simulink model "simulation_2"  (R2026a)
settings: Solver=VariableStepAuto  StopTime=10000
undefined symbols (not defined in the file): battery_builder_rtmsupport, gcbh
libraries: fl_lib x3, nesl_utility x3, BatteryCurrentManagement x1, Batteries_lib x1, BatteryEstimators x1
settings Model: Creator=dom  LastModifiedBy=dom

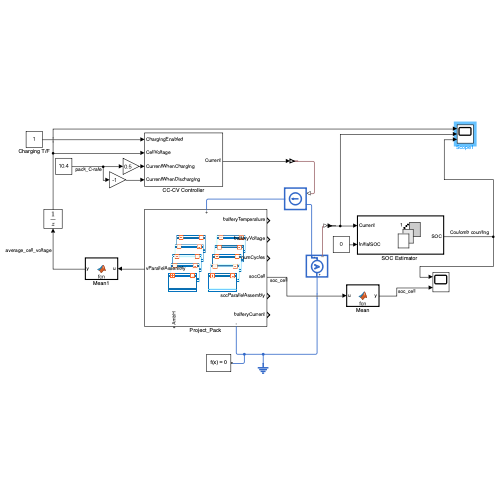
[thumbnail: Simulink's stored preview of the top-level diagram]
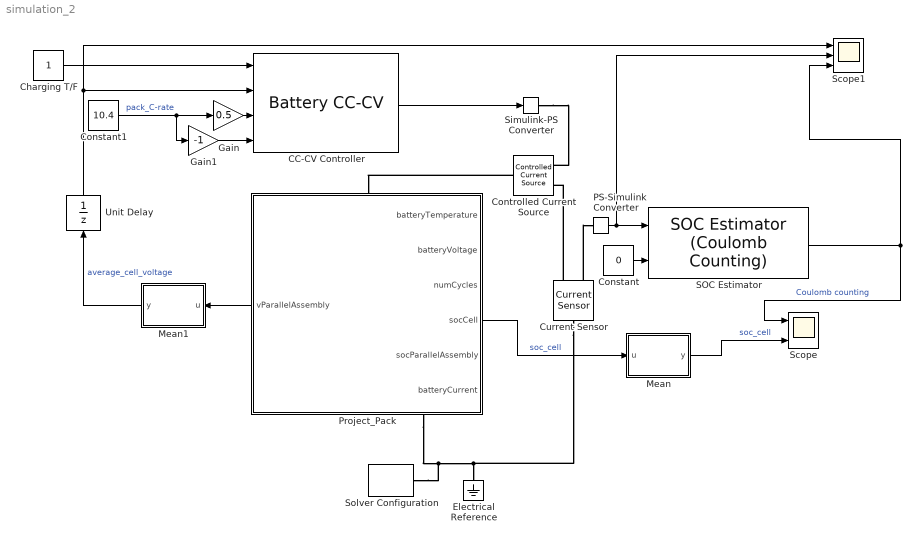
== system simulation_2 ==
  CC-CV Controller : BatteryCurrentManagement/Battery CC-CV  MinMaxFlag=off  MaxCellVoltage=4.2  Kp=100  Ki=10  Kaw=1  Kt=1  Ts=1
      settings: LibrarySourceBlock=batt_sl_lib/Current Management/Battery CC-CV
  Charging T/F : Constant
  Constant : Constant  Value=0
  Constant1 : Constant  Value=10.4
  Controlled Current Source : fl_lib/Electrical/Electrical Sources/Controlled Current Source
  Current Sensor : fl_lib/Electrical/Electrical Sensors/Current Sensor
  Electrical Reference : fl_lib/Electrical/Electrical Elements/Electrical Reference
  Gain : Gain  Gain=0.5
  Gain1 : Gain  Gain=-1
  Mean : MATLAB Function  TreatAsAtomicUnit=on
  Mean1 : MATLAB Function  TreatAsAtomicUnit=on
  PS-Simulink Converter : nesl_utility/PS-Simulink Converter  PhysicalDomain=network_engine_domain  SubClassName=ps_output  LeftPortType=input  RightPortType=output  PseudoPeriodic=off  Frequencies=[]  VectorFormat=inherit  Unit=inherit  AffineConversion=off
  Project_Pack : Subsystem  LoadFcn=battery_builder_rtmsupport('loadfcn',gcbh);
      settings: CopyFcn=battery_builder_rtmsupport('copyfcn',gcbh);  PreCopyFcn=battery_builder_rtmsupport('precopyfcn',gcbh);  PreDeleteFcn=battery_builder_rtmsupport('predeletefcn',gcbh);  PortSchema="{\"entries\":[{\"content\":{\"sides\":[{\"content\":{\"connectorIds\":[\"LConn1\"]},\"type\":\"ConnectorPlacement.EquallySpacedRectSide\",\"uuid\":\"76c6f046-db8e-4015-a922-00ba973faf16\"},{\"content\":{\"connectorIds\":[\"RConn1\",\"RConn2\"],\"side\":\"RIGHT\"},\"type\":\"ConnectorPlacement.EquallySpacedRectSide\",\"uuid\":\"59fdee5c-a6f4-4b44-aa6e-82d2d9418fce\"},{\"content\":{\"connectorIds\":[\"Out7\"],\"side\":\"TOP\"},\"type\":\"ConnectorPlacement.EquallySpacedRectSide\",\"uuid\":\"84b83595-cc1f-46da-a2b0-c16634a6daab\"},{\"content\":{\"connectorIds\":[\"Out1\",\"Out2\",\"Out3\",\"Out4\",\"Out5\",\"Out6\"],\"side\":\"BOTTOM\"},\"type\":\"ConnectorPlacement.EquallySpacedRectSide\",\"uuid\":\"4528fa0d-8164-4e66-baa6-2a345765de4f\"}]},\"type\":\"ConnectorPlacement.EquallySpacedConnector\",\"uuid\":\"e6fb231a-8daf-4bfc-bdc1-9175fa7a2dfd\"}],\"packageUris\":[\"http://schema.mathworks.com/mf0/Connector/R2020b\"],\"version\":\"1.0\"}"
      mask Display: image('$imagefile')
  "SOC Estimator " : BatteryEstimators/SOC Estimator (Coulomb Counting)  CurrentInputPartition=off  AH=10.4  Ts=1  DataType=Inherit: auto
      settings: LibrarySourceBlock=|
      | batt_sl_lib/Estimators/SOC Estimator
      | (Coulomb Counting)
  Scope : Scope  NumInputPorts=2
      settings: ActiveDisplayYMinimum=-0.12550450361997315  ActiveDisplayYMaximum=1.1295405325797585
  Scope1 : Scope  NumInputPorts=3
      settings: ActiveDisplayYMinimum=2.2867646550900531  ActiveDisplayYMaximum=4.4191181041895247
  Simulink-PS Converter : nesl_utility/Simulink-PS Converter  PhysicalDomain=network_engine_domain  SubClassName=ps_input  LeftPortType=input  RightPortType=output  PseudoPeriodic=off  Frequencies=[]  NoiseDistribution=none  NoiseParameters=[]  Unit=1  AffineConversion=off  FilteringAndDerivatives=provide  SimscapeFilterOrder=1  InputFilterTimeConstant=0.001  UdotUserProvided=0
  Solver Configuration : nesl_utility/Solver Configuration  PhysicalDomain=network_engine_domain  SubClassName=solver  LeftPortType=input  RightPortType=generic  Tones=[]  Harmonics=[]  SimulateNoise=off  Profile=off  UseLocalSampling=off  EnableSwitchedLinearOptims=on  FrequencyDomain=off  UseCCode=off  RelTol=0.001  AbsTol=0.001  MinStep=1e-09  ToWorkspace=off  RevertToSquareIcSolve=off  NumHomotopyIterations=100  PhasorMode=off  PhasorModeNumHarmonics=1  ConsistencySolver=NEWTON_XTOL_AFTER_FTOL  CanonicalOrdering=CANONICAL  OptimizeIntermediates=OPTIMIZED  IndexReductionMethod=DerivativeReplacement  DoDC=off  ResidualTolerance=1e-09  ConsistencyTolSource=GLOBAL  ConsistencyAbsTol=0.001  ConsistencyRelTol=0.001  ConsistencyTolFactor=0.001  UseLocalSolver=off  LocalSolverChoice=NE_BACKWARD_EULER_ADVANCER  ResolveIndetEquations=on  FunctionEvalNumThread=1  LocalSolverSampleTime=0.001  DoFixedCost=off  MaxNonlinIter=3  MaxModeIter=2  ComputeImpulses=off  ImpulseIterations=2  LinearAlgebra=auto  LinearAlgebraNumThread=0  EquationFormulation=NE_TIME_EF  DelaysMemoryBudget=1024  AutomaticFiltering=on  FilteringTimeConstant=0.001  PartitionStorageMethod=AS_NEEDED  PartitionMemoryBudget=1024  PartitionMethod=ROBUST  MultibodyUseLocalSolver=off  MultibodyLocalSolverChoice=ODE1  MultibodyLocalSolverSampleTime=0.001
  Unit Delay : UnitDelay  InitialCondition=2.5  SampleTime=-1
  wires:
  Project_Pack/4(socCell) -> Mean/1(u)  "soc_cell"
  Mean/1(y) -> Scope/2  "soc_cell"
  "SOC Estimator "/1 -> Scope/1, Scope1/3  "Coulomb counting"
  Constant/1 -> "SOC Estimator "/2
  PS-Simulink Converter/1 -> Scope1/2, "SOC Estimator "/1
  Gain/1 -> CC-CV Controller/3
  Project_Pack/7(vParallelAssembly) -> Mean1/1(u)
  Mean1/1(y) -> Unit Delay/1  "average_cell_voltage"
  Unit Delay/1 -> Scope1/1, CC-CV Controller/2
  Constant1/1 -> Gain/1, Gain1/1  "pack_C-rate"
  CC-CV Controller/1 -> Simulink-PS Converter/1
  Charging T/F/1 -> CC-CV Controller/1
  Gain1/1 -> CC-CV Controller/4
  connections:
  Project_Pack/RConn2 -- Current Sensor/LConn1 -- Electrical Reference/LConn1 -- Solver Configuration/RConn1
  Current Sensor/RConn1 -- PS-Simulink Converter/LConn1
  Simulink-PS Converter/RConn1 -- Controlled Current Source/RConn1
  Current Sensor/RConn2 -- Controlled Current Source/RConn2
  Controlled Current Source/LConn1 -- Project_Pack/LConn1

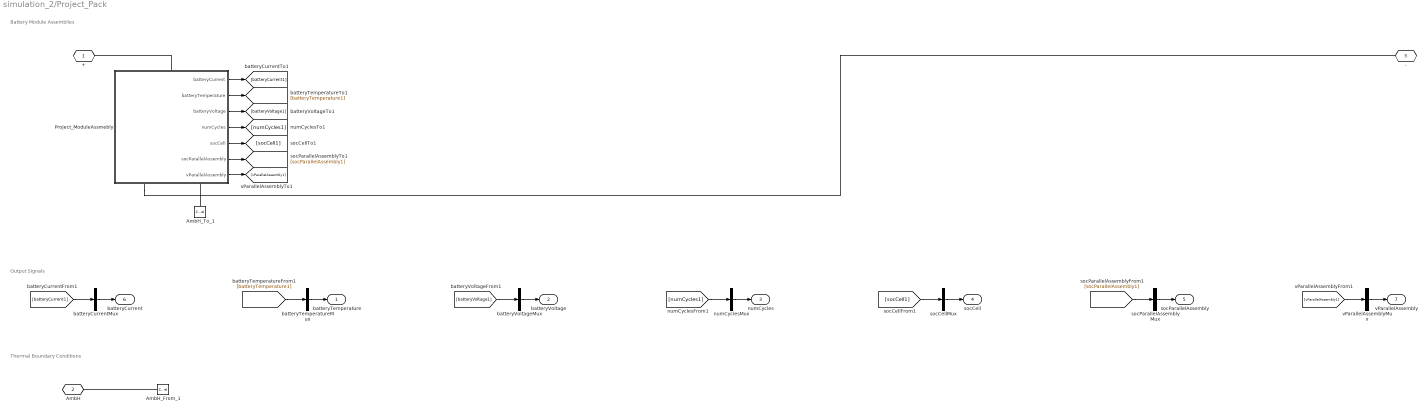
== system simulation_2/Project_Pack ==
  note: Thermal Boundary Conditions
  note: Output Signals
  note: Battery Module Assemblies
  AmbH_From_1 : ConnectionLabel  Label=ambH_1
  AmbH_To_1 : ConnectionLabel  Label=ambH_1
  Project_ModuleAssmebly : Subsystem  LoadFcn=battery_builder_rtmsupport('loadfcn',gcbh);
      settings: CopyFcn=battery_builder_rtmsupport('copyfcn',gcbh);  PreCopyFcn=battery_builder_rtmsupport('precopyfcn',gcbh);  PreDeleteFcn=battery_builder_rtmsupport('predeletefcn',gcbh);  PortSchema="{\"entries\":[{\"content\":{\"sides\":[{\"content\":{\"connectorIds\":[\"LConn1\"]},\"type\":\"ConnectorPlacement.EquallySpacedRectSide\",\"uuid\":\"76c6f046-db8e-4015-a922-00ba973faf16\"},{\"content\":{\"connectorIds\":[\"RConn1\",\"RConn2\"],\"side\":\"RIGHT\"},\"type\":\"ConnectorPlacement.EquallySpacedRectSide\",\"uuid\":\"59fdee5c-a6f4-4b44-aa6e-82d2d9418fce\"},{\"content\":{\"side\":\"TOP\"},\"type\":\"ConnectorPlacement.EquallySpacedRectSide\",\"uuid\":\"84b83595-cc1f-46da-a2b0-c16634a6daab\"},{\"content\":{\"connectorIds\":[\"Out1\",\"Out2\",\"Out3\",\"Out4\",\"Out5\",\"Out6\",\"Out7\"],\"side\":\"BOTTOM\"},\"type\":\"ConnectorPlacement.EquallySpacedRectSide\",\"uuid\":\"391f6102-8f79-4306-a331-0bb83eeeb4a2\"}]},\"type\":\"ConnectorPlacement.EquallySpacedConnector\",\"uuid\":\"e6fb231a-8daf-4bfc-bdc1-9175fa7a2dfd\"}],\"packageUris\":[\"http://schema.mathworks.com/mf0/Connector/R2020b\"],\"version\":\"1.0\"}"
      mask Display: image('$imagefile')
  batteryCurrentMux : Mux  Inputs=1
  batteryTemperatureMux : Mux  Inputs=1
  batteryVoltageMux : Mux  Inputs=1
  numCyclesMux : Mux  Inputs=1
  socCellMux : Mux  Inputs=1
  socParallelAssemblyMux : Mux  Inputs=1
  vParallelAssemblyMux : Mux  Inputs=1
  + : PMIOPort  Side=Left
  AmbH : PMIOPort  Port=2  Side=Right  ConnectionType=Connection: foundation.thermal.thermal
  - : PMIOPort  Port=3  Side=Right
  batteryTemperature : Outport
  batteryVoltage : Outport  Port=2
  numCycles : Outport  Port=3
  socCell : Outport  Port=4
  socParallelAssembly : Outport  Port=5
  batteryCurrent : Outport  Port=6
  vParallelAssembly : Outport  Port=7
  wires:
  [vParallelAssembly1] -> vParallelAssemblyMux/1
  vParallelAssemblyMux/1 -> vParallelAssembly/1
  Project_ModuleAssmebly/7(vParallelAssembly) -> [vParallelAssembly1]
  [socParallelAssembly1] -> socParallelAssemblyMux/1
  socParallelAssemblyMux/1 -> socParallelAssembly/1
  Project_ModuleAssmebly/6(socParallelAssembly) -> [socParallelAssembly1]
  [socCell1] -> socCellMux/1
  socCellMux/1 -> socCell/1
  Project_ModuleAssmebly/5(socCell) -> [socCell1]
  [numCycles1] -> numCyclesMux/1
  numCyclesMux/1 -> numCycles/1
  Project_ModuleAssmebly/4(numCycles) -> [numCycles1]
  [batteryVoltage1] -> batteryVoltageMux/1
  batteryVoltageMux/1 -> batteryVoltage/1
  Project_ModuleAssmebly/3(batteryVoltage) -> [batteryVoltage1]
  [batteryTemperature1] -> batteryTemperatureMux/1
  batteryTemperatureMux/1 -> batteryTemperature/1
  Project_ModuleAssmebly/2(batteryTemperature) -> [batteryTemperature1]
  [batteryCurrent1] -> batteryCurrentMux/1
  batteryCurrentMux/1 -> batteryCurrent/1
  Project_ModuleAssmebly/1(batteryCurrent) -> [batteryCurrent1]
  connections:
  AmbH_From_1/LConn1 -- AmbH/RConn1
  AmbH_To_1/LConn1 -- Project_ModuleAssmebly/RConn2
  Project_ModuleAssmebly/RConn1 -- -/RConn1
  Project_ModuleAssmebly/LConn1 -- +/RConn1

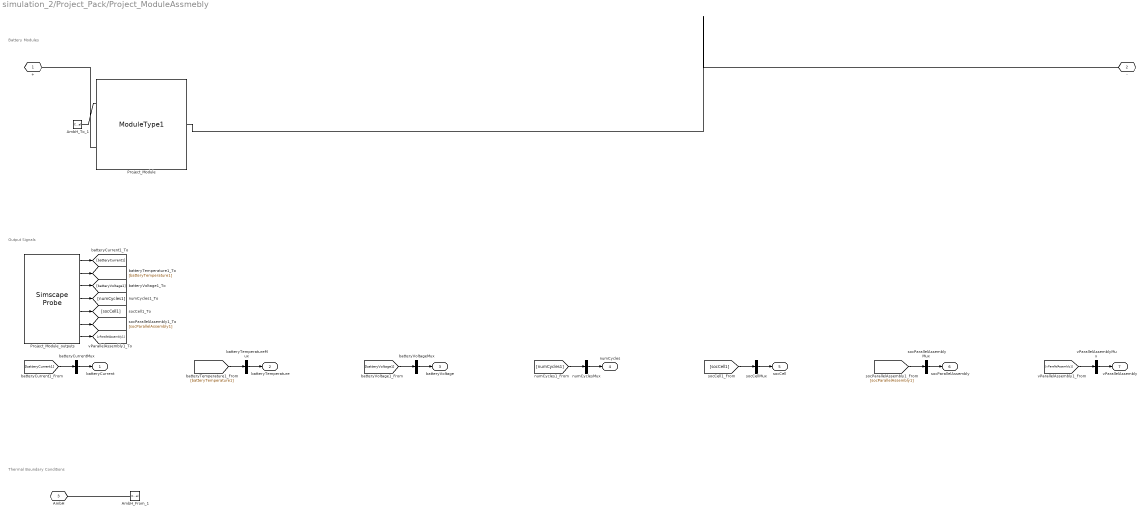
== system simulation_2/Project_Pack/Project_ModuleAssmebly ==
  note: Battery Modules
  note: Output Signals
  note: Thermal Boundary Conditions
  AmbH_From_1 : ConnectionLabel  Label=ambH_1
  AmbH_To_1 : ConnectionLabel  Label=ambH_1
  Project_Module : Batteries_lib/Modules/ModuleType1  BatteryCapacityCell=2.6 A*hr  ExtrapolationMethodCell=simscape.enum.extrapolation.nearest  SOCBreakpointsCell=[ 0 .1 .2 .3 .4 .5 .6 .7 .8 .9 1]  TemperatureBreakpointsCell=[273.15 293.15] K  OpenCircuitVoltageThermalCell=[2.5 2.5; 3 3; 3.2 3.2; 3.4 3.4; 3.5 3.5; 3.6 3.6;3.7 3.7;3.8 3.8;3.9 3.9;4 4;4.2 4.2] V  VoltageRangeCell=[0, inf] V  ResistanceSOCBreakpointsCell=[0, .1, .25, .5, .75, .9, 1]  ResistanceTemperatureBreakpointsCell=[278, 293, 313] K  R0ThermalCell=[.0117, .0085, .009; .011, .0085, .009; .0114, .0087, .0092; .0107, .0082, .0088; .0107, .0083, .0091; .0113, .0085, .0089; .0116, .0085, .0089] Ohm  BatteryThermalMassCell=100 J/K  AmbientResistance=25 K/W  socCell_specify=on  socCell_priority=High  socCell=0  socCell_nominal_specify=off  socCell_nominal_value=1  socCell_nominal_unit=1  batteryVoltage_specify=off  batteryVoltage_priority=None  batteryVoltage=0 V  batteryVoltage_nominal_specify=off  batteryVoltage_nominal_value=1  batteryVoltage_nominal_unit=V  batteryCurrent_specify=off  batteryCurrent_priority=None  batteryCurrent=0 A  batteryCurrent_nominal_specify=off  batteryCurrent_nominal_value=1  batteryCurrent_nominal_unit=A  numCycles_specify=off  numCycles_priority=High  numCycles=0  numCycles_nominal_specify=off  numCycles_nominal_value=1  numCycles_nominal_unit=1  batteryTemperature_specify=off  batteryTemperature_priority=High  batteryTemperature=298.15 K  batteryTemperature_nominal_specify=off  batteryTemperature_nominal_value=1  batteryTemperature_nominal_unit=K  vParallelAssembly_specify=off  vParallelAssembly_priority=None  vParallelAssembly=repmat(0, 10, 1) V  vParallelAssembly_nominal_specify=off  vParallelAssembly_nominal_value=1  vParallelAssembly_nominal_unit=V  socParallelAssembly_specify=off  socParallelAssembly_priority=None  socParallelAssembly=repmat(1, 10, 1)  socParallelAssembly_nominal_specify=off  socParallelAssembly_nominal_value=1  socParallelAssembly_nominal_unit=1
  Project_Module_outputs : SimscapeProbe  BoundBlock=482  Variables="{\"batteryCurrent\":{\"Probing\":\"ON\"},\"batteryTemperature\":{\"Probing\":\"ON\"},\"batteryVoltage\":{\"Probing\":\"ON\"},\"numCycles\":{\"Probing\":\"ON\"},\"socCell\":{\"Probing\":\"ON\"},\"socParallelAssembly\":{\"Probing\":\"ON\"},\"vParallelAssembly\":{\"Probing\":\"ON\"}}"
  batteryCurrentMux : Mux  Inputs=1
  batteryTemperatureMux : Mux  Inputs=1
  batteryVoltageMux : Mux  Inputs=1
  numCyclesMux : Mux  Inputs=1
  socCellMux : Mux  Inputs=1
  socParallelAssemblyMux : Mux  Inputs=1
  vParallelAssemblyMux : Mux  Inputs=1
  + : PMIOPort  Side=Left
  - : PMIOPort  Port=2  Side=Right
  AmbH : PMIOPort  Port=3  Side=Right  ConnectionType=Connection: foundation.thermal.thermal
  batteryCurrent : Outport
  batteryTemperature : Outport  Port=2
  batteryVoltage : Outport  Port=3
  numCycles : Outport  Port=4
  socCell : Outport  Port=5
  socParallelAssembly : Outport  Port=6
  vParallelAssembly : Outport  Port=7
  wires:
  Project_Module_outputs/1 -> [batteryCurrent1]
  batteryCurrentMux/1 -> batteryCurrent/1
  [batteryCurrent1] -> batteryCurrentMux/1
  Project_Module_outputs/2 -> [batteryTemperature1]
  batteryTemperatureMux/1 -> batteryTemperature/1
  [batteryTemperature1] -> batteryTemperatureMux/1
  Project_Module_outputs/3 -> [batteryVoltage1]
  batteryVoltageMux/1 -> batteryVoltage/1
  [batteryVoltage1] -> batteryVoltageMux/1
  Project_Module_outputs/4 -> [numCycles1]
  numCyclesMux/1 -> numCycles/1
  [numCycles1] -> numCyclesMux/1
  Project_Module_outputs/5 -> [socCell1]
  socCellMux/1 -> socCell/1
  [socCell1] -> socCellMux/1
  Project_Module_outputs/6 -> [socParallelAssembly1]
  socParallelAssemblyMux/1 -> socParallelAssembly/1
  [socParallelAssembly1] -> socParallelAssemblyMux/1
  Project_Module_outputs/7 -> [vParallelAssembly1]
  vParallelAssemblyMux/1 -> vParallelAssembly/1
  [vParallelAssembly1] -> vParallelAssemblyMux/1
  connections:
  Project_Module/LConn2 -- +/RConn1
  Project_Module/RConn1 -- -/RConn1
  AmbH_To_1/LConn1 -- Project_Module/LConn1
  AmbH_From_1/LConn1 -- AmbH/RConn1

== matlab function simulation_2/Mean ==
  data: u input; y output
function y = fcn(u)

y = mean(u);

end

== matlab function simulation_2/Mean1 ==
  data: u input; y output
function y = fcn(u)

y = mean(u);

end
